simulink model "step2_rf_link"  (R2026b)
settings: Solver=VariableStepAuto
libraries: commdigbbndpm3 x2, commchan3 x1, commrandsrc3 x1, commsink2 x1
settings Model: Creator=AYUSH  LastModifiedBy=AYUSH

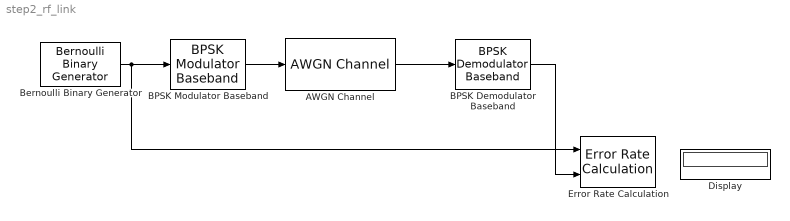
== system step2_rf_link ==
  AWGN Channel : commchan3/AWGN Channel  LegacyMode=off  NoiseMethod="Signal to noise ratio  (SNR)"  noiseMode="Signal to noise ratio  (SNR)"  EbNo=10  EsNo=10  SNR=rf_snr_db  BitsPerSymbol=1  SignalPower=1  SpecifySymbolPeriod=off  SamplesPerSymbol=1  SymbolPeriod=1  VarianceSource=Parameter  Variance=1  RandomStream=mt19937ar with seed  Seed=67  SimulateUsing=Code generation
  BPSK Demodulator Baseband : commdigbbndpm3/BPSK Demodulator Baseband  DecType=Hard decision  VarSource=Dialog  Variance=1  Ph=0  outDtype=Inherit via internal rule  derotateFactorWordLen=16  derotateFactorDataTypeStr=Inherit: Same word length as input  derotateFactorLastDataTypeStr=Inherit: Same word length as input
  BPSK Modulator Baseband : commdigbbndpm3/BPSK Modulator Baseband  Ph=0  outDtype=double  outWordLen=16  outUDDataType=sfix(16)  outFracLenMode=Best precision  outFracLen=15  outDataTypeStr=double  outLastDataTypeStr=double
  Bernoulli Binary Generator : commrandsrc3/Bernoulli Binary Generator  ProbabilityOfZero=0.5  SeedSource=Auto  Seed=12345  SampleTime=1  SamplesPerFrame=10000  OutputDataType=double  SimulateUsing=Interpreted execution
  Display : Display
  Error Rate Calculation : commsink2/Error Rate Calculation  N=0  st_delay=0  cp_mode=Entire frame  subframe=[]  PMode=Workspace  WsName=ber_result  RsMode2=off  stop=off  numErr=100  maxBits=1e6
  wires:
  Bernoulli Binary Generator/1 -> Error Rate Calculation/1, BPSK Modulator Baseband/1
  BPSK Modulator Baseband/1 -> AWGN Channel/1
  AWGN Channel/1 -> BPSK Demodulator Baseband/1
  BPSK Demodulator Baseband/1 -> Error Rate Calculation/2
